simulink model "robot_control_model"  (R2018b)
settings: Solver=ode45  StartTime=0.0  StopTime=12  MaxStep=p.dt  RelTol=1e-3
settings Model: Creator=leoni  LastModifiedBy=leoni

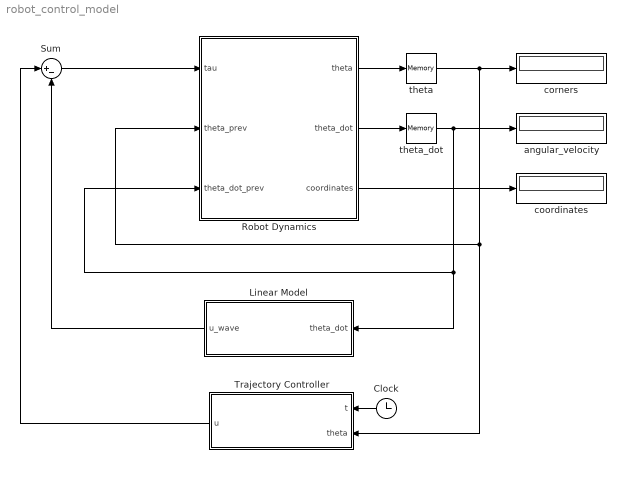
== system robot_control_model ==
  Clock : Clock
  Linear Model : MATLAB Function  TreatAsAtomicUnit=on
  Robot Dynamics : MATLAB Function  TreatAsAtomicUnit=on
  Sum : Sum  Inputs=|+-
  Trajectory Controller : MATLAB Function  TreatAsAtomicUnit=on
  angular_velocity : Display
  coordinates : Display
  corners : Display
  theta : Memory  InitialCondition=[0; pi/4; pi/3]
  theta_dot : Memory  InitialCondition=[0; 0; 0]
  wires:
  Sum/1 -> Robot Dynamics/1(tau)
  Robot Dynamics/1(theta) -> theta/1
  Robot Dynamics/2(theta_dot) -> theta_dot/1
  Robot Dynamics/3(coordinates) -> coordinates/1
  Clock/1 -> Trajectory Controller/1(t)
  theta/1 -> Robot Dynamics/2(theta_prev), Trajectory Controller/2(theta), corners/1
  theta_dot/1 -> Linear Model/1(theta_dot), Robot Dynamics/3(theta_dot_prev), angular_velocity/1
  Linear Model/1(u_wave) -> Sum/2
  Trajectory Controller/1(u) -> Sum/1

== matlab function robot_control_model/Linear Model ==
  data: theta_dot input; u_wave output
%Linear model of robot manipulator
function u_wave = linear_model(theta_dot)

    %p = robot_parameters();
    u_wave = p.K * theta_dot; %[3 x 3] * [3 x 1]
    
end

== matlab function robot_control_model/Trajectory Controller ==
  data: t input; u output; theta input
function u = trajectory_control(t, theta)
    
    %p = robot_parameters();
    JJ = jacobian_matrix(theta);
    [phi, Q] = phi_Q(t, theta);
    
    %regularization
    regular = 1e-6 * eye(3); 
    if any(isnan(JJ(:))) || any(isinf(JJ(:)))
        JJ = regular;
    end
    if any(isnan(phi(:))) || any(isinf(phi(:)))
        phi = [1e-6; 1e-6; 1e-6];
    end
        
    %u = [JJ*K^-1]^-1 * [alpha*phi - Q]
    %K^-1 = p.K
    u = (JJ * p.K) \ (p.alpha * phi - Q); %[3 x 3] \ [3 x 1]
    
end

== matlab function robot_control_model/Robot Dynamics ==
  data: tau input; theta output; theta_prev input; theta_dot_prev input; theta_dot output; coordinates output
%Model of robot manipulator
function [theta, theta_dot, coordinates] = robot_model(tau, theta_prev, theta_dot_prev)

    M = inertia_matrix(theta_prev, p);    
    h = coriolis_vector(theta_prev, theta_dot_prev, p);
    
    %regularization
    regular = 1e-6 * eye(3); 
    if any(isnan(M(:))) || any(isinf(M(:)))
        M = regular;
    end
    if any(isnan(h(:))) || any(isinf(h(:)))
        h = [1e-6; 1e-6; 1e-6];
    end
    
    friction = p.K * theta_dot_prev + p.F * sign(theta_dot_prev);
    theta_ddot = (p.J_0 + M) \ (tau - h - friction);
    
    theta_dot = theta_dot_prev + theta_ddot * p.dt; 
    theta = theta_prev + theta_dot * p.dt;
    
    [X, Y, Z] = forward_kinematics(theta, p);
    coordinates = [X, Y, Z];
   
end
